simulink model "Silmulink"  (R2023a)
settings: Solver=FixedStepAuto  StartTime=0.0  StopTime=2  FixedStep=0.001  RelTol=1e-3
PostLoadFcn:
  | LED;
  | load('DriveCycles.mat');
  | set_param(gcs,'StopTime',num2str(DrCycles.HWFET(end,1)));
settings Model: Creator=Qw011  LastModifiedBy=Qw011
settings OptimizationCC: DefaultParameterBehavior=Inlined  EnhancedBackFolding=on  PassReuseOutputArgsAs=Individual arguments  ZeroExternalMemoryAtStartup=off  ZeroInternalMemoryAtStartup=off  OptimizeBlockOrder=speed  DifferentSizesBufferReuse=on  OptimizationCustomize=off  EfficientTunableParamExpr=on
settings DebuggingCC: ParameterTunabilityLossMsg=error
settings SFSimCC: MATLABDynamicMemAlloc=off
settings RTWCC: Description=Embedded Coder  SystemTargetFile=ert.tlc  TemplateMakefile=ert_default_tmf
settings CodeAppCC: ForceParamTrailComments=on  IgnoreCustomStorageClasses=off  OperatorAnnotations=on  SimulinkDataObjDesc=on  SFDataObjDesc=on  InsertBlockDesc=on
settings ERTTargetCC: TargetLangStandard=C99 (ISO)  InlinedParameterPlacement=NonHierarchical  ERTCustomFileTemplate=example_file_process.tlc

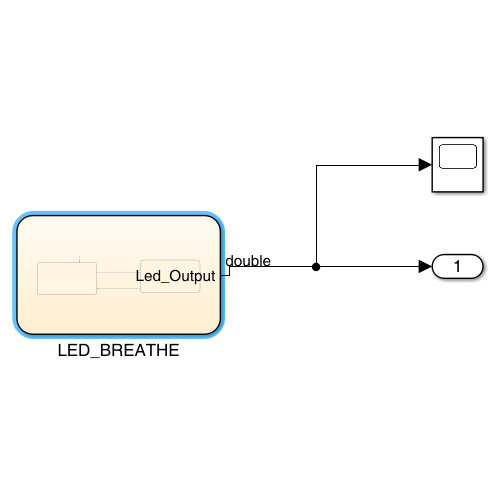
[thumbnail: Simulink's stored preview of the top-level diagram]
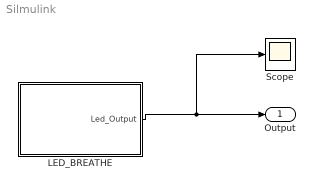
== system Silmulink ==
  LED_BREATHE : Stateflow chart  TreatAsAtomicUnit=on
  Scope : Scope
  Output : Outport
  wires:
  LED_BREATHE/1(Led_Output) -> Scope/1, Output/1

== stateflow chart Silmulink/LED_BREATHE ==
  state LedDark
    du:
    Led_Output=Led_Output - 1;
  state LedLight
    en:
    Led_Output=0;
    du:
    Led_Output = Led_Output + 1;
  (default) -> LedLight
  LedLight -> LedDark : [Led_Output >= 999]
  LedDark -> LedLight : [Led_Output <= 0]
  data: Led_Output output
